simulink model "bimanual_Diedrichsen"  (Simulink 8.1)
settings: Solver=ode4  SolverMode=SingleTasking  StartTime=0.0  StopTime=inf  FixedStep=0.0005  RelTol=1e-3
model workspace (MAT data in the model file):
  col_x = 1
  col_y = 2
  COL_VRAD = 3
  COL_LRAD = 4
  COL_FRAD = 5
  COL_COLOUR = 6
  COL_GOOD_COLOUR = 7
  COL_SLOW_COLOUR = 8
  COL_MISSED_COLOUR = 9
  COL_VY_ON_FX1 = 1
  COL_VY_ON_FX2 = 2
  COL_START_TARGET = 1
  COL_END_TARGET = 2
  COL_LOAD = 3
  COL_CURSOR_SELECTION = 4
  COL_1ST_TARGET_WAIT = 5
  COL_RANDOM_WAIT = 6
  COL_MAX_REACH_TIME = 7
  COL_2ND_TARGET_WAIT = 8
  COL_POST_TRIAL_DELAY = 9
  COL_HAND_FEEDBACK = 10
  E_STAY_CENTER = 2
  E_TARGET_ON = 3
  E_HOLD_AT_TARGET = 5
  E_HAND_FDBK_OFF = 11
  BKIN_STEP_TIME : num (value not decoded)
StartFcn:
  |  warndlg('Dexterit-E models cannot run under simulation. Please compile your model and run it from within Dexterit-E.');set_param(bdroot,'SimulationCommand','stop')
undefined symbols (not defined in the file or in its folder): slselsubs
libraries: Video x3, General x3, KINARM_EP_loads x3, KINARM_general x2, KINARM_loads x2, xpclib x1
(part 1 of 3)
CloseFcn:
  | rtwprivate ssgencode ModelCloseRequest b2lab2d
settings Model: Creator=Chris Grebeldinger  LastModifiedBy=dmclean  ModifiedComment=chris -- Wed Feb 16 09:18:30 2005 -- Version 1.1384  ModifiedHistory=Feb 16/05 - Add error repeat, add offset ramp  ExtModeArmWhenConnect=off  ExtModeLogAll=off  BufferReuse=off
settings DataIOCC: LimitDataPoints=off  SaveOutput=off  SaveTime=off  SignalLoggingName=sigsOut
settings OptimizationCC: BlockReduction=off  BooleanDataType=off  OptimizeBlockIOStorage=off  BufferReuse=off  ExpressionFolding=off  FoldNonRolledExpr=off  LocalBlockOutputs=off  InitFltsAndDblsToZero=on
settings DebuggingCC: SaveWithParameterizedLinksMsg=none  SignalResolutionControl=TryResolveAllWithWarning  SolverPrmCheckMsg=none  MultiTaskDSMMsg=warning  MultiTaskCondExecSysMsg=none  StrictBusMsg=None
settings HardwareCC: ProdIntDivRoundTo=Zero  ProdEndianess=LittleEndian  ProdHWDeviceType=Generic->32-bit x86 compatible  TargetHWDeviceType=32-bit Generic
settings SFSimCC: SimParseCustomCode=off
settings RTWCC: SystemTargetFile=xpctarget.tlc  TemplateMakefile=xpc_default_tmf  Description=xPC Target  ProcessScript=xpctarget_make_rtw_hook  IncludeERTFirstTime=on  RTWCompilerOptimization=On
settings CodeAppCC: MaxIdLength=63
settings xpcTargetCC: TargetFcnLib=ansi_tfl_tmw.mat  CodeReplacementLibrary=XPC_BLAS  ParMdlRefBuildCompliant=on  ConcurrentExecutionCompliant=on  CombineSignalStateStructs=off  MATLABClassNameForMDSCustomization=xpcAperiodicCustomization  GRTInterface=on  GenerateAllocFcn=off  xPCTaskExecutionProfile=off  xPCRL32EventNumber=5000  xPCisDownloadable=off  xPCLoadParamSetFile=off  xPCConcurrentTasks=off  xPCEnableSFAnimation=off

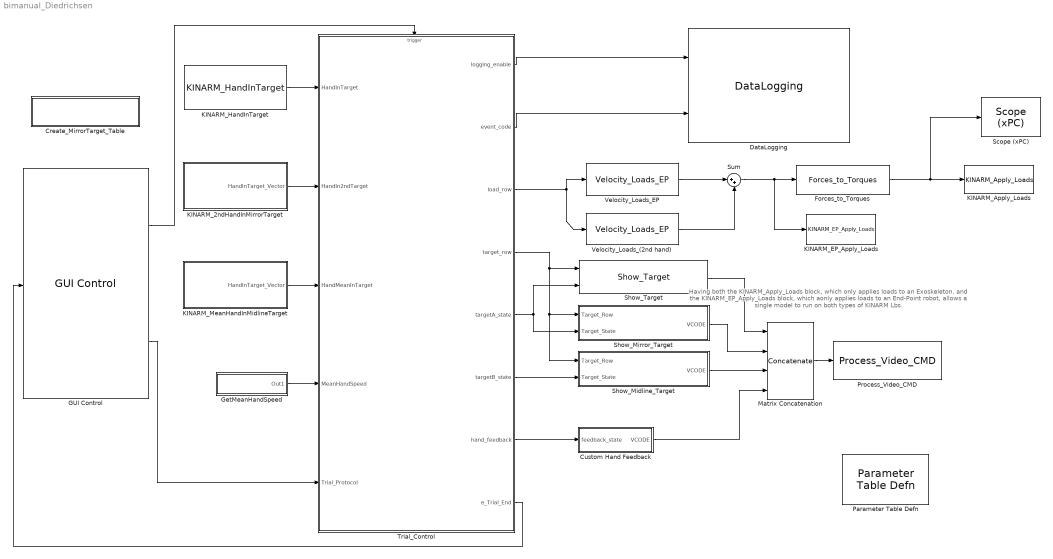
== system bimanual_Diedrichsen ==
  note: Having both the KINARM_Apply_Loads block, which only
      | applies loads to an Exoskeleton, and the KINARM_EP_Apply_Loads
      |  block, which aonly applies loads to an End-Point robot, allows
      | a single model to run on both types of KINARM Lbs.
  Create_MirrorTarget_Table : Subsystem
  Custom Hand Feedback : Subsystem
  DataLogging : General/DataLogging  log_event_codes=on  log_analog_inputs=off
      link override Poll KINARM/EPTorqueCMD: GotoTag=KINARMEPTorqueCMD
      link override Poll KINARM/TorqueCMD: GotoTag=KINARMTorqueCMD
  Forces_to_Torques : KINARM_loads/Forces_to_Torques
  GUI Control : General/GUI Control  target_type_str=Circle  Target_Type=1  XYcols=[1 2]  Vcols=3  Lcols=4  indices_padding=[0 0 0 0;0 0 0 0]  task_version=1.0  show_repeat_trial_flag=off
  GetMeanHandSpeed : Subsystem
  KINARM_2ndHandInMirrorTarget : Subsystem  AncestorBlock=KINARM_general/KINARM_HandInTarget  mask(KINARM_HandInTarget){use_dominant_hand=off, target_type=Circle, num_states=1, attribcol1=4, attribcol2=4, attribcol3=5, attribcol4=6}
      mask prompts: use_dominant_hand "Dominant Hand?"; target_type "Type of Target"; num_states "Number of Target States"; attribcol1 "State 1 Target Table Column(s)"; attribcol2 "State 2 Target Table Column(s)"; attribcol3 "State 3 Target Table Column(s)"; attribcol4 "State 4 Target Table Column(s)"
      mask help: This block returns a vector or array corresponding to the Target_Table rows indicating whether the specified hand is in (=1) or out (=0) of each of the targets.
      mask init:
      | num_states=str2num(get_param(gcb, 'num_states'));
      | columntext='(columns: ';
      | 
      | for i=1:num_states
      | 	varname=['attribcol' num2str(i)];
      | 	if i>1
      | 		columntext=[columntext, '; '];
      | 	end
      | 	columntext=[columntext, get_param(gcb, varname)];
      | end
      | columntext=strvcat([columntext ')'],' ', ' ');
      | 
      | output_block=char(find_system(gcb,'LookUnderMasks','all','FollowLinks','on','SearchDepth',1,'BlockType','Outport'));
      | outputname=get_param(output_block,'Name');
      | 
      | % Select only the desired states for output. The output port is also renamed to reflect 
      | % whether the output is a vector (in the case of a single state) or an array (of vectors, 
      | % one for each of multiple states).
      | if num_states == 1
      | 	set_param([gcb '/Selected States'], 'Value', '[1]');
      | 	set_param(output_block, 'Name', 'HandInTarget_Vector');
      | elseif num_states == 2
      | 	set_param([gcb '/Selected States'], 'Value', '[1,2]');
      | 	set_param(output_block, 'Name', 'HandInTarget_Array');
      | elseif num_states == 3
      | 	set_param([gcb '/Selected States'], 'Value', '[1,2,3]');
      | 	set_param(output_block, 'Name', 'HandInTarget_Array');
      | else
      | 	set_param([gcb '/Selected States'], 'Value', '[1,2,3,4]');
      | 	set_param(output_block, 'Name', 'HandInTarget_Array');
      | end
      mask Help:
      | Used to determine if the hand (finger-tip) is in any of the targets in the Target_Table.
      | <P>
      | <B><I>Use of this block requires that the DataLogging block (General library) be set to log KINARM data.</I></B>
      | 
      | <H2>Library </H2>
      | KINARM_general (sub-library)
      | 
      | <H2>Description </H2>
      | This block returns a vector or array corresponding to the Target_Table rows indicating whether the specified hand (i.e. finger-tip) is in or out of each of the targets.  Each element in the output vector or output array will be either a 0 (hand not in target) or a 1 (hand in target).
      | <P>
      | A vector is returned if only one target state is specified in each target row (see Parameters and Dialog Box), with each index of the vector corresponding to a row in the target table.  An array is returned if more than one target state is specified in a target row, with each row of the array corresponding to a target row and each column corresponding to the nth target state specified in each target row.
      | <P>
      | The output vector or array is typically used by a stateflow chart to affect behavior of the system.  Because this block returns hand-in-target information for all targets in the target table, multiple targets can be monitored at once (i.e. the stateflow chart could have certain transitions that occur if the hand is in one target and other transitions if it is in a different target).  Likewise, because this block returns hand-in-target information for multiple states of a single target, those multiple states can be monitored simultaneously.
      | <P>
      | Because the KINARM_HandInTarget block returns information for only one hand, two copies of this block are required if information for both hands is desired.
      | <P>
      | 
      | <H2>Parameters and Dialog Box</H2>
      | <B>Dominant Hand?:</B> this box determines which hand is used by this block : dominant hand position (checked box) or the non-dominant hand position (unchecked box).  (Note: if the end-user wants to know about both the dominant hand and the non-dominant hand, then 2 separate copies of this block are requried, one for each hand.)
      | <P>
      | <B>Type of Target:</B> Enter the type of target specified in the target table:
      | <P>
      | <B>Number of Target States:</B> Enter the number of target states specified in each target row.  Up to four target states are allowed per target row.
      | <P>
      | <B>State <n> Target Table Columns:</B> Enter the columns in the Target Table that specify the relevant target attributes.  Do this for each target state.
      | For a circle, enter the columns corresponding to logical radius (e.g. 4)
      | <BR>For an ellipse, enter the columns corresponding to major radius, minor radius, rotation angle (e.g. [4, 5, 6]).
      | <BR>For a rectangle, enter the columns corresponding to length, height, and rotation angle (e.g. [4, 5, 6]).
      | <BR>For a line, enter the columns corresponding to stroke width, endpoint in x, and endpoint in y (e.g. [3, 4, 5]).
      | <BR>For a triangle, enter the columns corresponding to length, height, peak offset, and rotation angle (e.g. [4, 5, 6, 7]).
      | 
      | <H2>Examples</H2>
      | <B>Example 1.</B>  Suppose a target row will be used to define 1 state for a circle type target and the radius of the visual target is the same radius to be used for determination of hand-in-target.  The related Target Table column is: column 6 = radius.  For this example, "State 1 Target Table Columns" would equal [6].
      | <P>
      | 
      | <B>Example 2.</B>  Suppose a target row will be used to define 1 state for a circle type target, but the radius of the visual target will be different than the radius to be used for determination of hand-in-target.  This option allows independent control over the size of the visual target versus the accuracy needed to be considered "in the target".  The related Target Table columns are: column 6 = radius1 (i.e. radius to target to be drawn); column 7 = radius2 (i.e. radius to be used for hand-in-target) .  For this example, "State 1 Target Table Columns" would equal [7].
      | <P>
      | <B>Example 3.</B>  Suppose a target row will be used to define 2 states for a circle type target, where the radius of the visual target will be a constant, but depending on the state of the system, one of 2 other and different radii will be used for determination of hand-in-target.  The related Target Table columns are: column 6 = radius1 (i.e. radius to target to be drawn); column 7 = radius2 (i.e. radius to be used for hand-in-target for state 1); column 8 = radius3 (i.e. radius to be used for hand-in-target for state 2).  For this example, "State 1 Target Table Columns" would equal [7], while "State 2 Target Table Columns" would equal [8].
      | <P>
      | 
      | <H2>Related Blocks </H2>
      | DataLogging
      mask TypeOptions target_type: Circle | Ellipse | Rectangle | Line | Triangle
      mask Callback target_type:
      | target_type=get_param(gcb, 'target_type');
      | attribcol1=[str2num(get_param(gcb, 'attribcol1')) 0 0 0 0 0 0];
      | attribcol2=[str2num(get_param(gcb, 'attribcol2')) 0 0 0 0 0 0];
      | attribcol3=[str2num(get_param(gcb, 'attribcol3')) 0 0 0 0 0 0];
      | attribcol4=[str2num(get_param(gcb, 'attribcol4')) 0 0 0 0 0 0];
      | switch target_type(1:3)
      | 	case 'Cir'
      | 		numcol=1;
      | 	case 'Ell'
      | 		numcol=3;
      |     case 'Rec'
      |         numcol=3;
      |     case 'Lin'
      |         numcol=3;
      |     case 'Tri'
      |         numcol=4;
      | 	otherwise
      | 		numcol=1;
      | end
      | if numcol==1
      | 	set_param(gcb, 'attribcol1', num2str(attribcol1(1)));
      | 	set_param(gcb, 'attribcol2', num2str(attribcol2(1)));
      | 	set_param(gcb, 'attribcol3', num2str(attribcol3(1)));
      | 	set_param(gcb, 'attribcol4', num2str(attribcol4(1)));
      | else
      | 	set_param(gcb, 'attribcol1', ['[' num2str(attribcol1(1:numcol)) ']']);
      | 	set_param(gcb, 'attribcol2', ['[' num2str(attribcol2(1:numcol)) ']']);
      | 	set_param(gcb, 'attribcol3', ['[' num2str(attribcol3(1:numcol)) ']']);
      | 	set_param(gcb, 'attribcol4', ['[' num2str(attribcol4(1:numcol)) ']']);
      | end
      mask TypeOptions num_states: 1 | 2 | 3 | 4
      mask Callback num_states:
      | num_states = str2num(get_param(gcb, 'num_states'));
      | vis = get_param(gcb, 'MaskVisibilities');
      | 
      | % Select only the desired states for output. The output port is also renamed to reflect
      | % whether the output is a vector (in the case of a single state) or an array (of vectors,
      | % one for each of multiple states).
      | output_block=char(find_system(gcb, 'LookUnderMasks', 'all', 'FollowLinks', 'on', 'SearchDepth', 1, 'BlockType', 'Outport'));
      | 
      | if num_states == 1
      | 	set_param([gcb '/Selected States'], 'Value', '[1]');
      | 	set_param(output_block, 'Name', 'HandInTarget_Vector');
      | 	vis{5} = 'off';
      | 	vis{6} = 'off';
      | 	vis{7} = 'off';
      | elseif num_states == 2
      | 	set_param([gcb '/Selected States'], 'Value', '[1,2]');
      | 	set_param(output_block, 'Name', 'HandInTarget_Array');
      | 	vis{5} = 'on';
      | 	vis{6} = 'off';
      | 	vis{7} = 'off';
      | elseif num_states == 3
      | 	set_param([gcb '/Selected States'], 'Value', '[1,2,3]');
      | 	set_param(output_block, 'Name','HandInTarget_Array');
      | 	vis{5} = 'on';
      | 	vis{6} = 'on';
      | 	vis{7} = 'off';
      | else
      | 	set_param([gcb '/Selected States'], 'Value', '[1,2,3,4]');
      | 	set_param(output_block, 'Name', 'HandInTarget_Array');
      | 	vis{5} = 'on';
      | 	vis{6} = 'on';
      | 	vis{7} = 'on';
      | end
      | set_param(gcb, 'MaskVisibilities', vis);
      | 
      | target_type=get_param(gcb, 'target_type');
      | attribcol1=[str2num(get_param(gcb, 'attribcol1')) 0 0 0 0 0 0];
      | attribcol2=[str2num(get_param(gcb, 'attribcol2')) 0 0 0 0 0 0];
      | attribcol3=[str2num(get_param(gcb, 'attribcol3')) 0 0 0 0 0 0];
      | attribcol4=[str2num(get_param(gcb, 'attribcol4')) 0 0 0 0 0 0];
      | switch target_type(1:3)
      | 	case 'Cir'
      | 		numcol=1;
      | 	case 'Ell'
      | 		numcol=3;
      |     case 'Rec'
      |         numcol=3;
      |     case 'Lin'
      |         numcol=3;
      |     case 'Tri'
      |         numcol=4;
      | 	otherwise
      | 		numcol=1;
      | end
      | if numcol==1
      | 	set_param(gcb, 'attribcol1', num2str(attribcol1(1)));
      | 	set_param(gcb, 'attribcol2', num2str(attribcol2(1)));
      | 	set_param(gcb, 'attribcol3', num2str(attribcol3(1)));
      | 	set_param(gcb, 'attribcol4', num2str(attribcol4(1)));
      | else
      | 	set_param(gcb, 'attribcol1', ['[' num2str(attribcol1(1:numcol)) ']']);
      | 	set_param(gcb, 'attribcol2', ['[' num2str(attribcol2(1:numcol)) ']']);
      | 	set_param(gcb, 'attribcol3', ['[' num2str(attribcol3(1:numcol)) ']']);
      | 	set_param(gcb, 'attribcol4', ['[' num2str(attribcol4(1:numcol)) ']']);
      | end
      mask Callback attribcol1:
      | target_type=get_param(gcb, 'target_type');
      | attribcol1=[str2num(get_param(gcb, 'attribcol1')) 0 0 0 0 0 0];
      | attribcol2=[str2num(get_param(gcb, 'attribcol2')) 0 0 0 0 0 0];
      | attribcol3=[str2num(get_param(gcb, 'attribcol3')) 0 0 0 0 0 0];
      | attribcol4=[str2num(get_param(gcb, 'attribcol4')) 0 0 0 0 0 0];
      | switch target_type(1:3)
      | 	case 'Cir'
      | 		numcol=1;
      | 	case 'Ell'
      | 		numcol=3;
      |     case 'Rec'
      |         numcol=3;
      |     case 'Lin'
      |         numcol=3;
      |     case 'Tri'
      |         numcol=4;
      | 	otherwise
      | 		numcol=1;
      | end
      | if numcol==1
      | 	set_param(gcb, 'attribcol1', num2str(attribcol1(1)));
      | 	set_param(gcb, 'attribcol2', num2str(attribcol2(1)));
      | 	set_param(gcb, 'attribcol3', num2str(attribcol3(1)));
      | 	set_param(gcb, 'attribcol4', num2str(attribcol4(1)));
      | else
      | 	set_param(gcb, 'attribcol1', ['[' num2str(attribcol1(1:numcol)) ']']);
      | 	set_param(gcb, 'attribcol2', ['[' num2str(attribcol2(1:numcol)) ']']);
      | 	set_param(gcb, 'attribcol3', ['[' num2str(attribcol3(1:numcol)) ']']);
      | 	set_param(gcb, 'attribcol4', ['[' num2str(attribcol4(1:numcol)) ']']);
      | end
      mask Callback attribcol2:
      | target_type=get_param(gcb, 'target_type');
      | attribcol1=[str2num(get_param(gcb, 'attribcol1')) 0 0 0 0 0 0];
      | attribcol2=[str2num(get_param(gcb, 'attribcol2')) 0 0 0 0 0 0];
      | attribcol3=[str2num(get_param(gcb, 'attribcol3')) 0 0 0 0 0 0];
      | attribcol4=[str2num(get_param(gcb, 'attribcol4')) 0 0 0 0 0 0];
      | switch target_type(1:3)
      | 	case 'Cir'
      | 		numcol=1;
      | 	case 'Ell'
      | 		numcol=3;
      |     case 'Rec'
      |         numcol=3;
      |     case 'Lin'
      |         numcol=3;
      |     case 'Tri'
      |         numcol=4;
      | 	otherwise
      | 		numcol=1;
      | end
      | if numcol==1
      | 	set_param(gcb, 'attribcol1', num2str(attribcol1(1)));
      | 	set_param(gcb, 'attribcol2', num2str(attribcol2(1)));
      | 	set_param(gcb, 'attribcol3', num2str(attribcol3(1)));
      | 	set_param(gcb, 'attribcol4', num2str(attribcol4(1)));
      | else
      | 	set_param(gcb, 'attribcol1', ['[' num2str(attribcol1(1:numcol)) ']']);
      | 	set_param(gcb, 'attribcol2', ['[' num2str(attribcol2(1:numcol)) ']']);
      | 	set_param(gcb, 'attribcol3', ['[' num2str(attribcol3(1:numcol)) ']']);
      | 	set_param(gcb, 'attribcol4', ['[' num2str(attribcol4(1:numcol)) ']']);
      | end
      mask Callback attribcol3:
      | target_type=get_param(gcb, 'target_type');
      | attribcol1=[str2num(get_param(gcb, 'attribcol1')) 0 0 0 0 0 0];
      | attribcol2=[str2num(get_param(gcb, 'attribcol2')) 0 0 0 0 0 0];
      | attribcol3=[str2num(get_param(gcb, 'attribcol3')) 0 0 0 0 0 0];
      | attribcol4=[str2num(get_param(gcb, 'attribcol4')) 0 0 0 0 0 0];
      | switch target_type(1:3)
      | 	case 'Cir'
      | 		numcol=1;
      | 	case 'Ell'
      | 		numcol=3;
      |     case 'Rec'
      |         numcol=3;
      |     case 'Lin'
      |         numcol=3;
      |     case 'Tri'
      |         numcol=4;
      | 	otherwise
      | 		numcol=1;
      | end
      | if numcol==1
      | 	set_param(gcb, 'attribcol1', num2str(attribcol1(1)));
      | 	set_param(gcb, 'attribcol2', num2str(attribcol2(1)));
      | 	set_param(gcb, 'attribcol3', num2str(attribcol3(1)));
      | 	set_param(gcb, 'attribcol4', num2str(attribcol4(1)));
      | else
      | 	set_param(gcb, 'attribcol1', ['[' num2str(attribcol1(1:numcol)) ']']);
      | 	set_param(gcb, 'attribcol2', ['[' num2str(attribcol2(1:numcol)) ']']);
      | 	set_param(gcb, 'attribcol3', ['[' num2str(attribcol3(1:numcol)) ']']);
      | 	set_param(gcb, 'attribcol4', ['[' num2str(attribcol4(1:numcol)) ']']);
      | end
      mask Callback attribcol4:
      | target_type=get_param(gcb, 'target_type');
      | attribcol1=[str2num(get_param(gcb, 'attribcol1')) 0 0 0 0 0 0];
      | attribcol2=[str2num(get_param(gcb, 'attribcol2')) 0 0 0 0 0 0];
      | attribcol3=[str2num(get_param(gcb, 'attribcol3')) 0 0 0 0 0 0];
      | attribcol4=[str2num(get_param(gcb, 'attribcol4')) 0 0 0 0 0 0];
      | switch target_type(1:3)
      | 	case 'Cir'
      | 		numcol=1;
      | 	case 'Ell'
      | 		numcol=3;
      |     case 'Rec'
      |         numcol=3;
      |     case 'Lin'
      |         numcol=3;
      |     case 'Tri'
      |         numcol=4;
      | 	otherwise
      | 		numcol=1;
      | end
      | if numcol==1
      | 	set_param(gcb, 'attribcol1', num2str(attribcol1(1)));
      | 	set_param(gcb, 'attribcol2', num2str(attribcol2(1)));
      | 	set_param(gcb, 'attribcol3', num2str(attribcol3(1)));
      | 	set_param(gcb, 'attribcol4', num2str(attribcol4(1)));
      | else
      | 	set_param(gcb, 'attribcol1', ['[' num2str(attribcol1(1:numcol)) ']']);
      | 	set_param(gcb, 'attribcol2', ['[' num2str(attribcol2(1:numcol)) ']']);
      | 	set_param(gcb, 'attribcol3', ['[' num2str(attribcol3(1:numcol)) ']']);
      | 	set_param(gcb, 'attribcol4', ['[' num2str(attribcol4(1:numcol)) ']']);
      | end
      mask Display:
      | disp(columntext)
      | port_label('output',1,outputname)
  KINARM_Apply_Loads : KINARM_loads/KINARM_Apply_Loads  up_duration=50  down_duration=50  max_torque=13
  KINARM_EP_Apply_Loads : KINARM_EP_loads/KINARM_EP_Apply_Loads  up_duration=1500  down_duration=1500  max_force=60
  KINARM_HandInTarget : KINARM_general/KINARM_HandInTarget  use_dominant_hand=on  target_type=Circle  num_states=1  attribcol1=[4]  attribcol2=[4]  attribcol3=[5]  attribcol4=[6]  attribcol5=[0]
  KINARM_MeanHandInMidlineTarget : Subsystem  AncestorBlock=KINARM_general/KINARM_HandInTarget  mask(KINARM_HandInTarget){use_dominant_hand=off, target_type=Circle, num_states=1, attribcol1=4, attribcol2=4, attribcol3=5, attribcol4=6}
      mask prompts: use_dominant_hand "Dominant Hand?"; target_type "Type of Target"; num_states "Number of Target States"; attribcol1 "State 1 Target Table Column(s)"; attribcol2 "State 2 Target Table Column(s)"; attribcol3 "State 3 Target Table Column(s)"; attribcol4 "State 4 Target Table Column(s)"
      mask help: This block returns a vector or array corresponding to the Target_Table rows indicating whether the specified hand is in (=1) or out (=0) of each of the targets.
      mask init: same as bimanual_Diedrichsen/KINARM_2ndHandInMirrorTarget
      mask Help:
      | Used to determine if the hand (finger-tip) is in any of the targets in the Target_Table.
      | <P>
      | <B><I>Use of this block requires that the DataLogging block (General library) be set to log KINARM data.</I></B>
      | 
      | <H2>Library </H2>
      | KINARM_general (sub-library)
      | 
      | <H2>Description </H2>
      | This block returns a vector or array corresponding to the Target_Table rows indicating whether the specified hand (i.e. finger-tip) is in or out of each of the targets.  Each element in the output vector or output array will be either a 0 (hand not in target) or a 1 (hand in target).
      | <P>
      | A vector is returned if only one target state is specified in each target row (see Parameters and Dialog Box), with each index of the vector corresponding to a row in the target table.  An array is returned if more than one target state is specified in a target row, with each row of the array corresponding to a target row and each column corresponding to the nth target state specified in each target row.
      | <P>
      | The output vector or array is typically used by a stateflow chart to affect behavior of the system.  Because this block returns hand-in-target information for all targets in the target table, multiple targets can be monitored at once (i.e. the stateflow chart could have certain transitions that occur if the hand is in one target and other transitions if it is in a different target).  Likewise, because this block returns hand-in-target information for multiple states of a single target, those multiple states can be monitored simultaneously.
      | <P>
      | Because the KINARM_HandInTarget block returns information for only one hand, two copies of this block are required if information for both hands is desired.
      | <P>
      | 
      | <H2>Parameters and Dialog Box</H2>
      | <B>Dominant Hand?:</B> this box determines which hand is used by this block : dominant hand position (checked box) or the non-dominant hand position (unchecked box).  (Note: if the end-user wants to know about both the dominant hand and the non-dominant hand, then 2 separate copies of this block are requried, one for each hand.)
      | <P>
      | <B>Type of Target:</B> Enter the type of target specified in the target table:
      | <P>
      | <B>Number of Target States:</B> Enter the number of target states specified in each target row.  Up to four target states are allowed per target row.
      | <P>
      | <B>State <n> Target Table Columns:</B> Enter the columns in the Target Table that specify the relevant target attributes.  Do this for each target state.
      | For a circle, enter the columns corresponding to logical radius (e.g. 4)
      | <BR>For an ellipse, enter the columns corresponding to major radius, minor radius, rotation angle (e.g. [4, 5, 6]).
      | <BR>For a rectangle, enter the columns corresponding to length, height, and rotation angle (e.g. [4, 5, 6]).
      | <BR>For a line, enter the columns corresponding to stroke width, endpoint in x, and endpoint in y (e.g. [3, 4, 5]).
      | <BR>For a triangle, enter the columns corresponding to length, height, peak offset, and rotation angle (e.g. [4, 5, 6, 7]).
      | 
      | <H2>Examples</H2>
      | <B>Example 1.</B>  Suppose a target row will be used to define 1 state for a circle type target and the radius of the visual target is the same radius to be used for determination of hand-in-target.  The related Target Table column is: column 6 = radius.  For this example, "State 1 Target Table Columns" would equal [6].
      | <P>
      | 
      | <B>Example 2.</B>  Suppose a target row will be used to define 1 state for a circle type target, but the radius of the visual target will be different than the radius to be used for determination of hand-in-target.  This option allows independent control over the size of the visual target versus the accuracy needed to be considered "in the target".  The related Target Table columns are: column 6 = radius1 (i.e. radius to target to be drawn); column 7 = radius2 (i.e. radius to be used for hand-in-target) .  For this example, "State 1 Target Table Columns" would equal [7].
      | <P>
      | <B>Example 3.</B>  Suppose a target row will be used to define 2 states for a circle type target, where the radius of the visual target will be a constant, but depending on the state of the system, one of 2 other and different radii will be used for determination of hand-in-target.  The related Target Table columns are: column 6 = radius1 (i.e. radius to target to be drawn); column 7 = radius2 (i.e. radius to be used for hand-in-target for state 1); column 8 = radius3 (i.e. radius to be used for hand-in-target for state 2).  For this example, "State 1 Target Table Columns" would equal [7], while "State 2 Target Table Columns" would equal [8].
      | <P>
      | 
      | <H2>Related Blocks </H2>
      | DataLogging
      mask TypeOptions target_type: Circle | Ellipse | Rectangle | Line | Triangle
      mask Callback target_type:
      | target_type=get_param(gcb, 'target_type');
      | attribcol1=[str2num(get_param(gcb, 'attribcol1')) 0 0 0 0 0 0];
      | attribcol2=[str2num(get_param(gcb, 'attribcol2')) 0 0 0 0 0 0];
      | attribcol3=[str2num(get_param(gcb, 'attribcol3')) 0 0 0 0 0 0];
      | attribcol4=[str2num(get_param(gcb, 'attribcol4')) 0 0 0 0 0 0];
      | switch target_type(1:3)
      | 	case 'Cir'
      | 		numcol=1;
      | 	case 'Ell'
      | 		numcol=3;
      |     case 'Rec'
      |         numcol=3;
      |     case 'Lin'
      |         numcol=3;
      |     case 'Tri'
      |         numcol=4;
      | 	otherwise
      | 		numcol=1;
      | end
      | if numcol==1
      | 	set_param(gcb, 'attribcol1', num2str(attribcol1(1)));
      | 	set_param(gcb, 'attribcol2', num2str(attribcol2(1)));
      | 	set_param(gcb, 'attribcol3', num2str(attribcol3(1)));
      | 	set_param(gcb, 'attribcol4', num2str(attribcol4(1)));
      | else
      | 	set_param(gcb, 'attribcol1', ['[' num2str(attribcol1(1:numcol)) ']']);
      | 	set_param(gcb, 'attribcol2', ['[' num2str(attribcol2(1:numcol)) ']']);
      | 	set_param(gcb, 'attribcol3', ['[' num2str(attribcol3(1:numcol)) ']']);
      | 	set_param(gcb, 'attribcol4', ['[' num2str(attribcol4(1:numcol)) ']']);
      | end
      mask TypeOptions num_states: 1 | 2 | 3 | 4
      mask Callback num_states:
      | num_states = str2num(get_param(gcb, 'num_states'));
      | vis = get_param(gcb, 'MaskVisibilities');
      | 
      | % Select only the desired states for output. The output port is also renamed to reflect
      | % whether the output is a vector (in the case of a single state) or an array (of vectors,
      | % one for each of multiple states).
      | output_block=char(find_system(gcb, 'LookUnderMasks', 'all', 'FollowLinks', 'on', 'SearchDepth', 1, 'BlockType', 'Outport'));
      | 
      | if num_states == 1
      | 	set_param([gcb '/Selected States'], 'Value', '[1]');
      | 	set_param(output_block, 'Name', 'HandInTarget_Vector');
      | 	vis{5} = 'off';
      | 	vis{6} = 'off';
      | 	vis{7} = 'off';
      | elseif num_states == 2
      | 	set_param([gcb '/Selected States'], 'Value', '[1,2]');
      | 	set_param(output_block, 'Name', 'HandInTarget_Array');
      | 	vis{5} = 'on';
      | 	vis{6} = 'off';
      | 	vis{7} = 'off';
      | elseif num_states == 3
      | 	set_param([gcb '/Selected States'], 'Value', '[1,2,3]');
      | 	set_param(output_block, 'Name','HandInTarget_Array');
      | 	vis{5} = 'on';
      | 	vis{6} = 'on';
      | 	vis{7} = 'off';
      | else
      | 	set_param([gcb '/Selected States'], 'Value', '[1,2,3,4]');
      | 	set_param(output_block, 'Name', 'HandInTarget_Array');
      | 	vis{5} = 'on';
      | 	vis{6} = 'on';
      | 	vis{7} = 'on';
      | end
      | set_param(gcb, 'MaskVisibilities', vis);
      | 
      | target_type=get_param(gcb, 'target_type');
      | attribcol1=[str2num(get_param(gcb, 'attribcol1')) 0 0 0 0 0 0];
      | attribcol2=[str2num(get_param(gcb, 'attribcol2')) 0 0 0 0 0 0];
      | attribcol3=[str2num(get_param(gcb, 'attribcol3')) 0 0 0 0 0 0];
      | attribcol4=[str2num(get_param(gcb, 'attribcol4')) 0 0 0 0 0 0];
      | switch target_type(1:3)
      | 	case 'Cir'
      | 		numcol=1;
      | 	case 'Ell'
      | 		numcol=3;
      |     case 'Rec'
      |         numcol=3;
      |     case 'Lin'
      |         numcol=3;
      |     case 'Tri'
      |         numcol=4;
      | 	otherwise
      | 		numcol=1;
      | end
      | if numcol==1
      | 	set_param(gcb, 'attribcol1', num2str(attribcol1(1)));
      | 	set_param(gcb, 'attribcol2', num2str(attribcol2(1)));
      | 	set_param(gcb, 'attribcol3', num2str(attribcol3(1)));
      | 	set_param(gcb, 'attribcol4', num2str(attribcol4(1)));
      | else
      | 	set_param(gcb, 'attribcol1', ['[' num2str(attribcol1(1:numcol)) ']']);
      | 	set_param(gcb, 'attribcol2', ['[' num2str(attribcol2(1:numcol)) ']']);
      | 	set_param(gcb, 'attribcol3', ['[' num2str(attribcol3(1:numcol)) ']']);
      | 	set_param(gcb, 'attribcol4', ['[' num2str(attribcol4(1:numcol)) ']']);
      | end
      mask Callback attribcol1:
      | target_type=get_param(gcb, 'target_type');
      | attribcol1=[str2num(get_param(gcb, 'attribcol1')) 0 0 0 0 0 0];
      | attribcol2=[str2num(get_param(gcb, 'attribcol2')) 0 0 0 0 0 0];
      | attribcol3=[str2num(get_param(gcb, 'attribcol3')) 0 0 0 0 0 0];
      | attribcol4=[str2num(get_param(gcb, 'attribcol4')) 0 0 0 0 0 0];
      | switch target_type(1:3)
      | 	case 'Cir'
      | 		numcol=1;
      | 	case 'Ell'
      | 		numcol=3;
      |     case 'Rec'
      |         numcol=3;
      |     case 'Lin'
      |         numcol=3;
      |     case 'Tri'
      |         numcol=4;
      | 	otherwise
      | 		numcol=1;
      | end
      | if numcol==1
      | 	set_param(gcb, 'attribcol1', num2str(attribcol1(1)));
      | 	set_param(gcb, 'attribcol2', num2str(attribcol2(1)));
      | 	set_param(gcb, 'attribcol3', num2str(attribcol3(1)));
      | 	set_param(gcb, 'attribcol4', num2str(attribcol4(1)));
      | else
      | 	set_param(gcb, 'attribcol1', ['[' num2str(attribcol1(1:numcol)) ']']);
      | 	set_param(gcb, 'attribcol2', ['[' num2str(attribcol2(1:numcol)) ']']);
      | 	set_param(gcb, 'attribcol3', ['[' num2str(attribcol3(1:numcol)) ']']);
      | 	set_param(gcb, 'attribcol4', ['[' num2str(attribcol4(1:numcol)) ']']);
      | end
      mask Callback attribcol2:
      | target_type=get_param(gcb, 'target_type');
      | attribcol1=[str2num(get_param(gcb, 'attribcol1')) 0 0 0 0 0 0];
      | attribcol2=[str2num(get_param(gcb, 'attribcol2')) 0 0 0 0 0 0];
      | attribcol3=[str2num(get_param(gcb, 'attribcol3')) 0 0 0 0 0 0];
      | attribcol4=[str2num(get_param(gcb, 'attribcol4')) 0 0 0 0 0 0];
      | switch target_type(1:3)
      | 	case 'Cir'
      | 		numcol=1;
      | 	case 'Ell'
      | 		numcol=3;
      |     case 'Rec'
      |         numcol=3;
      |     case 'Lin'
      |         numcol=3;
      |     case 'Tri'
      |         numcol=4;
      | 	otherwise
      | 		numcol=1;
      | end
      | if numcol==1
      | 	set_param(gcb, 'attribcol1', num2str(attribcol1(1)));
      | 	set_param(gcb, 'attribcol2', num2str(attribcol2(1)));
      | 	set_param(gcb, 'attribcol3', num2str(attribcol3(1)));
      | 	set_param(gcb, 'attribcol4', num2str(attribcol4(1)));
      | else
      | 	set_param(gcb, 'attribcol1', ['[' num2str(attribcol1(1:numcol)) ']']);
      | 	set_param(gcb, 'attribcol2', ['[' num2str(attribcol2(1:numcol)) ']']);
      | 	set_param(gcb, 'attribcol3', ['[' num2str(attribcol3(1:numcol)) ']']);
      | 	set_param(gcb, 'attribcol4', ['[' num2str(attribcol4(1:numcol)) ']']);
      | end
      mask Callback attribcol3:
      | target_type=get_param(gcb, 'target_type');
      | attribcol1=[str2num(get_param(gcb, 'attribcol1')) 0 0 0 0 0 0];
      | attribcol2=[str2num(get_param(gcb, 'attribcol2')) 0 0 0 0 0 0];
      | attribcol3=[str2num(get_param(gcb, 'attribcol3')) 0 0 0 0 0 0];
      | attribcol4=[str2num(get_param(gcb, 'attribcol4')) 0 0 0 0 0 0];
      | switch target_type(1:3)
      | 	case 'Cir'
      | 		numcol=1;
      | 	case 'Ell'
      | 		numcol=3;
      |     case 'Rec'
      |         numcol=3;
      |     case 'Lin'
      |         numcol=3;
      |     case 'Tri'
      |         numcol=4;
      | 	otherwise
      | 		numcol=1;
      | end
      | if numcol==1
      | 	set_param(gcb, 'attribcol1', num2str(attribcol1(1)));
      | 	set_param(gcb, 'attribcol2', num2str(attribcol2(1)));
      | 	set_param(gcb, 'attribcol3', num2str(attribcol3(1)));
      | 	set_param(gcb, 'attribcol4', num2str(attribcol4(1)));
      | else
      | 	set_param(gcb, 'attribcol1', ['[' num2str(attribcol1(1:numcol)) ']']);
      | 	set_param(gcb, 'attribcol2', ['[' num2str(attribcol2(1:numcol)) ']']);
      | 	set_param(gcb, 'attribcol3', ['[' num2str(attribcol3(1:numcol)) ']']);
      | 	set_param(gcb, 'attribcol4', ['[' num2str(attribcol4(1:numcol)) ']']);
      | end
      mask Callback attribcol4:
      | target_type=get_param(gcb, 'target_type');
      | attribcol1=[str2num(get_param(gcb, 'attribcol1')) 0 0 0 0 0 0];
      | attribcol2=[str2num(get_param(gcb, 'attribcol2')) 0 0 0 0 0 0];
      | attribcol3=[str2num(get_param(gcb, 'attribcol3')) 0 0 0 0 0 0];
      | attribcol4=[str2num(get_param(gcb, 'attribcol4')) 0 0 0 0 0 0];
      | switch target_type(1:3)
      | 	case 'Cir'
      | 		numcol=1;
      | 	case 'Ell'
      | 		numcol=3;
      |     case 'Rec'
      |         numcol=3;
      |     case 'Lin'
      |         numcol=3;
      |     case 'Tri'
      |         numcol=4;
      | 	otherwise
      | 		numcol=1;
      | end
      | if numcol==1
      | 	set_param(gcb, 'attribcol1', num2str(attribcol1(1)));
      | 	set_param(gcb, 'attribcol2', num2str(attribcol2(1)));
      | 	set_param(gcb, 'attribcol3', num2str(attribcol3(1)));
      | 	set_param(gcb, 'attribcol4', num2str(attribcol4(1)));
      | else
      | 	set_param(gcb, 'attribcol1', ['[' num2str(attribcol1(1:numcol)) ']']);
      | 	set_param(gcb, 'attribcol2', ['[' num2str(attribcol2(1:numcol)) ']']);
      | 	set_param(gcb, 'attribcol3', ['[' num2str(attribcol3(1:numcol)) ']']);
      | 	set_param(gcb, 'attribcol4', ['[' num2str(attribcol4(1:numcol)) ']']);
      | end
      mask Display:
      | disp(columntext)
      | port_label('output',1,outputname)
  Matrix Concatenation : Concatenate  NumInputs=4  Mode=Multidimensional array
  Parameter Table Defn : General/Parameter Table Defn  ShowInLibBrowser=0
  Process_Video_CMD : Video/Process_Video_CMD
  "Scope (xPC) " : xpclib/Misc./Scope (xPC)   scopeno=1  scopetype=Target  autostart=on  viewmode=Numerical  formatstr='%15.6f'  grid=on  ylimits=[0,0]  nosamples=250  noprepostsamples=0  interleave=1  triggermode=FreeRun  triggersignal=1  trigsignalfromport=off  triggerlevel=0.0  triggerslope=Either  triggerscope=1  triggersample=0  filename=data.dat  mode=Lazy  writesize=512  autorestart=off  dynamicfilemode=off  maxwritefilesize=512*1024^2
  Show_Midline_Target : Subsystem  AncestorBlock=Video/Show_Target  mask(Show_Target){target_type=Circle, num_states=1, attribcol1=[6 6 0 3], attribcol2=[6 6 0 3], attribcol3=[7 7 0 3], attribcol4=[8 8 0 3], attribcol5=[0 0 24 0], stateindices_padding=[0 0 0 0 0 0 0;0 0 0 0 0 0 0;0 0 0 0 0 0 0;0 0 0 0 0 0 0;0 0 0 0 0 0 0], source=internal, opacity=100, target_display=Both subject and operator displays}
      mask prompts: target_type "Type of Target"; num_states "Number of Target States"; attribcol1 "State 1 Target Table Column(s)"; attribcol2 "State 2 Target Table Column(s)"; attribcol3 "State 3 Target Table Column(s)"; attribcol4 "State 4 Target Table Column(s)"; attribcol5 "State 5 Target Table Column(s)"; stateindices_padding "State Indices Padding"; source "Source for Opacity"; target_display "Target Display"
      mask help: This block returns a VCODE that, when sent to the Process_Video_CMD block, will cause a single target to be drawn. Target parameters are specified in the Target Table according to the columns defined below and the row input to this block.
      mask init:
      | block_path = gcb;  % store block path, as gcb may change with block operations
      | 
      | % Handle background colours if link status changes.  If the link is resolved, 
      | % make the block back to the library colour.  If the link is not resolved, 
      | % change the colour to something other than the library block colour (but 
      | % only change it if it is the library colour, that way end-users can choose
      | % their own colour.
      | link_status = get_param(block_path, 'LinkStatus');
      | block_parent = get_param(block_path, 'Parent');
      | if strcmp(link_status, 'resolved') || strcmp(block_parent, 'Video')
      | 	set_param(block_path, 'BackgroundColor', '[0.85882, 0.69019, 0.3098]');
      | else
      |  	current_bgcolor = str2num( get_param(block_path, 'BackgroundColor') ) ;
      | 	%if the BackgroundColor is 'green', then after the str2num, current_bgcolor is empty
      | 	if ~isempty(current_bgcolor) 
      | 		if (round(current_bgcolor * 255) == [219 176 79])
      | 	 		set_param(block_path, 'BackgroundColor', 'green');
      | 		end
      | 	end
      | end
      | 
      | num_states=str2num(get_param(gcb, 'num_states'));
      | columntext='';
      | 
      | for i=1:num_states
      | 	varname=['attribcol' num2str(i)];
      | 	if i>1
      | 		columntext=strvcat(columntext, get_param(gcb, varname));
      | 	else
      | 		columntext=[get_param(gcb, varname)];
      | 	end
      | end
      | 
      | space=[''];
      | n=round(length(columntext)/2)-4;
      | for i=1:n
      | 	space=[space ' '];
      | end
      | columntext=strvcat([space '(columns)'], columntext);
      | 
      | output_block=char(find_system(gcb,'LookUnderMasks','all','FollowLinks','on','SearchDepth',1,'BlockType','Outport'));
      | outputname=get_param(output_block,'Name');
      | input_block=find_system(gcb,'LookUnderMasks','all','FollowLinks','on','SearchDepth',1,'BlockType','Inport');
      | inputname1=get_param(char(input_block{1}),'Name');
      | inputname2=get_param(char(input_block{2}),'Name');
      | 
      | if length(input_block) >= 3
      |     inputname3=get_param(char(input_block{3}),'Name');
      | end
      | 
      | source=get_param(gcb,'source');
      | vis=get_param(gcb,'MaskVisibilities');
      | num_states=str2num(get_param(gcb, 'num_states'));
      | 
      | if source=='internal'
      | 	if length(input_block) == 3
      | 		pos=get_param([gcb '/Opacity'],'position');
      | 		delete_line(gcb, 'Opacity/1', 'Embedded MATLAB Function/4');
      | 		delete_block(input_block{3});
      |         add_block('built-in/Constant',[gcb '/Opacity'],'Name','Opacity');
      | 		set_param([gcb '/Opacity'],'position',pos);
      | 		add_line(gcb, 'Opacity/1', 'Embedded MATLAB Function/4');
      | 		set_param([gcb '/Opacity'],'Value','opacity');
      | 	end
      | 	displaytext = ['disp(columntext); port_label(''output'',1,outputname); port_label(''input'',1, inputname1); port_label(''input'',2, inputname2);'];
      | 	vis{10}='on';
      | else
      | 	if length(input_block) == 2
      | 		pos=get_param([gcb '/Opacity'],'position');
      | 		delete_line(gcb, 'Opacity/1', 'Embedded MATLAB Function/4');
      | 		delete_block([gcb, '/Opacity']);
      | 		add_block('built-in/Inport',[gcb '/In2'],'Name','Opacity');
      | 		set_param([gcb '/Opacity'],'position',pos);
      | 		add_line(gcb, 'Opacity/1', 'Embedded MATLAB Function/4');
      |  	end
      | 	inputname3='Opacity';
      | 	displaytext = ['disp(columntext); port_label(''output'',1,outputname); port_label(''input'',1, inputname1); port_label(''input'',2, inputname2); port_label(''input'',3, inputname3);'];
      | 	vis{10}='off';
      | end
      | 
      | targetDisplay = get_param(gcb,'target_display');
      | 
      | if length(targetDisplay) == length('Subject display only')
      |     set_param([gcb '/Target_Display'], 'Value', '2');
      | elseif length(targetDisplay) == length('Operator display only')
      |     set_param([gcb '/Target_Display'], 'Value', '3');
      | else
      |     set_param([gcb '/Target_Display'], 'Value', '1');
      | end
      |     
      | set_param(gcb,'MaskVisibilities',vis);
      | set_param(gcb,'MaskDisplay',displaytext);
      mask Help:
      | Used to draw a single, stationary target.
      | 
      | <H2>Library </H2>
      | Video
      | 
      | <H2>Description </H2>
      | This block returns a VCODE, which when sent to the Process_Video_CMD block will draw a single stationary target.  The VCODE contains all of the target parameters necessary to draw the target.
      | <P>
      | The VCODE is generated from information contained in the Target Table.  Which parts of the Target Table are used depends on the columns selected (see Parameters and Dialog Box below)<P>
      | 
      | <p>For example, assume the "row" input is 2, the "type of target" is set to "Circle" and the "Target Table Columns" is set to [3 0 0 4]. Then using the sample target table below a red circle will be drawn at (20cm, 40cm) and have a radius of 2cm. The zeros in the  "Target Table Columns" indicate those parameters are not used.
      | 
      | <tt>
      | _____________________________________________<br>
      | |&nbsp;&nbsp;&nbsp;&nbsp;&nbsp;&nbsp;&nbsp;&nbsp;&nbsp;&nbsp;| X Pos | Y pos |&nbsp;&nbsp;Fill | Radius |<br>
      | ---------------------------------------------<br>
      | | target 1 |&nbsp;&nbsp;&nbsp;&nbsp;10 |&nbsp;&nbsp;&nbsp;&nbsp;10 | white |&nbsp;&nbsp;&nbsp;&nbsp;&nbsp;&nbsp;5 |<br>
      | | target 2 |&nbsp;&nbsp;&nbsp;&nbsp;20 |&nbsp;&nbsp;&nbsp;&nbsp;40 |&nbsp;&nbsp;&nbsp;red |&nbsp;&nbsp;&nbsp;&nbsp;&nbsp;&nbsp;2 |<br>
      | | target 3 |&nbsp;&nbsp;&nbsp;-40 |&nbsp;&nbsp;&nbsp;&nbsp;10 |&nbsp;&nbsp;blue |&nbsp;&nbsp;&nbsp;&nbsp;&nbsp;&nbsp;3 |<br>
      | ---------------------------------------------<br>
      | </tt>
      | <p> Inputs:<br>
      | <B> Target_Row: </B> this scalar input determines which row in the Target Table is used to define the target parameters.  Typically the Target_Row comes from the Trial_Protocol.  <P>
      | <B> Target_State: </B> this scalar input determines which state the Target is in.  Different states reference different columns in the Target Table (as defined in the Dialog Box).  Typically the Target_State is controlled by the Stateflow_chart to dynamically change the appearance of the target depending on system and/or subject behavior.  Target_State=0 is a valid input, which turns the target off (the intended method for turning a target off is to set Target_State=0). <BR>
      | <P>
      | There is one output from this block:
      | <P>
      | <B> VCODE: </B> this output is a vector containing one VCODE.  This output must go to the Process_Video_CMD block of the video library for the target to actually be shown (if any other visual targets are to be displayed, then this VCODE output must be concatenated with the other VCODES prior to connection to the Process_Video_CMD block - see Help for the Process_Video_CMD block for more information).
      | <P>
      | To show multiple targets simultaneously, multiple copies of the Show_Target block can be used in a Task Program.  The output VCODES from multiple Show_Target blocks must be concatenated prior to connection to the Process_Video_CMD block.
      | <P>
      | 
      | <H2>Parameters and Dialog Box</H2>
      | <B>Type of Target:</B> Choose the type of target specified in the target table.
      | <P>
      | <B>Number of Target States:</B> Choose the number of target states specified in each target row.  Up to five target states are allowed per target row.
      | <P>
      | <B>State [n] Target Table Columns:</B> Enter the column indices that specify the relevant target attributes in the Target Table.  All target types have the same first three target attributes: fill colour, stroke colour and stroke width.
      | <Blockquote>
      | <P>
      | Element 1 (fill colour) - points to the column index in the Target Table containing the fill colour.  If this index is 0, then the fill colour is transparent and the Target Table is not referenced.  For line targets, the fill colour is not used.
      | <P>
      | Element 2 (stroke colour) - points to the column index in the Target Table containing the stroke colour.  If this index is 0, then the stroke colour is transparent and the Target Table is not referenced.  It is possible to use the same column index for both fill colour and stroke colour (i.e.  if single-colour targets are desired).  For line targets, stroke colour defines the colour of the line.
      | <P>
      | Element 3 (stroke width) - points to the column index in the Target Table containing the stroke width (cm).  If no stroke is desired, then setting the stroke column index to 0 will produce a stroke width of 0  and the Target Table is not referenced.  Setting stroke column index to a value less than;0 will produce a standard 1 mm stroke width, again without referencing the Target Table.  For line targets, stroke width defines the width of the line.
      | <P>
      | <B><I>Circle</I></B> <P>
      | Element 4 (radius) - radius of the circle (cm).
      | <P>
      | <B><I>Ellipse</I></B> <P>
      | Elements 4-6 (ellipse properties) - major radius (cm), minor radius (cm), rotation angle (degrees).  If no rotation is desired, then setting rotation column index to 0 will produce a default rotation of 0 and the Target Table will not be referenced.
      | <P>
      | <B><I>Rectangle</I></B><P>
      | Elements 4-6 (rectangle properties) - length (cm), height (cm), rotation angle (degrees).  If no rotation is desired, then setting rotation column index to 0 will produce a default rotation of 0 and the Target Table will not be referenced.
      | <P>
      | <B><I>Line</I></B><P>
      | Elements 4-5 (line properties) - end point x-axis position relative to start point (cm), end point y-axis position relative to start point (cm). The width and colour of the line are defined by the stroke width and the stroke colour, respectively.  The fill colour column is ignored (i.e. any value can be used for column 1)
      | <P>
      | <B><I>Triangle</I></B><P>
      | Elements 4-7 (triangle properties) - length (cm), height (cm), offset of peak of triangle relative to midpoint of the length (cm), rotation angle (degrees). If a height column index of 0 is specified, then an equilateral triangle with sides of the specified length will be created and the Target Table will not be referenced for height or peak offset.  If no rotation is desired, then setting a rotation column index of 0 will produce a default rotation of 0 and the Target Table will not be referenced.
      | </Blockquote>
      | <P>
      | Each target state requires its own set of column index definitions (although multiple states can point to the same column index if desired).<P>
      | <H2>Examples</H2>
      | <B>Example 1.</B>  Suppose a target row will be used to define 2 states for a circle type target.  The first state will be a solid circle of colour1 and the second state will be identical, except that it will have colour2.  The related Target Table columns are: column 4 = colour1; column 5 = colour2 and column 6 = radius.  For this example, "State 1 Target Table Columns" would equal [4 4 0 6], while "State 2 Target Table Columns" would equal [5 5 0 6].  In other words, the fill and stroke colours are both taken from the same column of the Target Table, and there is no outside stroke.
      | <P>
      | 
      | <B>Example 2.</B>  Suppose a target row will be used to define 2 states for an circle type target.  The first state will have fill colour "colour1" and stroke colour "colour2" and radius "rad1".  The second state will have fill colour "colour3" and stroke colour "colour2" and radius "rad2".  Both states will have stroke width "str_width".  The related Target Table columns are: column4 = colour1; column 5 = colour2; column 6 = colour3; column 7 = str_width; column 8 = rad1; column 9 = rad2.  For this example, "State 1 Target Table Columns" would equal [4 5 7 8], while "State 2 Target Table Columns" would equal [6 5 7 9].
      | <P>
      | 
      | <B>Example 3.</B>  Suppose a target row will be used to define 1 state for an ellipse type target.  It will be an outline ellipse with a stroke colour but no fill colour and a standard 1mm stroke width.  The related Target Table columns are: column 4 = colour; column 5 = major radius; column 6 = minor radius and column 7 = orientation.  For this example, "State 1 Target Table Columns" would equal [0 4 -1 5 6 7].
      | <P>
      | 
      | <H2>Related Blocks </H2>
      | Show_Target_With_Label<BR>
      | Process_Video_CMD
      mask TypeOptions target_type: Circle | Ellipse | Rectangle | Line | Triangle
      mask Callback target_type:
      | target_type=get_param(gcb, 'target_type');
      | attribcol1=[str2num(get_param(gcb, 'attribcol1')) 0 0 0 0 0 0];
      | attribcol2=[str2num(get_param(gcb, 'attribcol2')) 0 0 0 0 0 0];
      | attribcol3=[str2num(get_param(gcb, 'attribcol3')) 0 0 0 0 0 0];
      | attribcol4=[str2num(get_param(gcb, 'attribcol4')) 0 0 0 0 0 0];
      | attribcol5=[str2num(get_param(gcb, 'attribcol5')) 0 0 0 0 0 0];
      | switch target_type(1:3)
      | 	case 'Cir'
      | 		numcol=4;
      | 	case 'Ell'
      | 		numcol=6;
      |     case 'Rec'
      |         numcol=6;
      |     case 'Lin'
      |         numcol=5;
      |     case 'Tri'
      |         numcol=7;
      |     otherwise
      | 		numcol=4;
      | end
      | set_param(gcb, 'attribcol1', mat2str(attribcol1(1:numcol)));
      | set_param(gcb, 'attribcol2', mat2str(attribcol2(1:numcol)));
      | set_param(gcb, 'attribcol3', mat2str(attribcol3(1:numcol)));
      | set_param(gcb, 'attribcol4', mat2str(attribcol4(1:numcol)));
      | set_param(gcb, 'attribcol5', mat2str(attribcol5(1:numcol)));
      | 
      | stateindices_padding=zeros(5,7);
      | set_param(gcb, 'stateindices_padding', mat2str(stateindices_padding(:, 1:(11-numcol))));
      mask TypeOptions num_states: 1 | 2 | 3 | 4 | 5
      mask Callback num_states:
      | main_block=gcb;
      | num_states=str2num(get_param(main_block, 'num_states'));
      | vis=get_param(main_block,'MaskVisibilities');
      | 
      | %If the number of states>1, then output an array instead of a vector.
      | %Only show those inputs necessary on the Mask
      | output_block=char(find_system(gcb,'LookUnderMasks','all','SearchDepth',1,'BlockType','Outport'));
      | if num_states==1			%output of HandInTarget block is a vector
      | 	vis{4}='off';
      | 	vis{5}='off';
      | 	vis{6}='off';
      | 	vis{7}='off';
      | elseif num_states==2					%output of HandInTarget block is an array
      | 	vis{4}='on';
      | 	vis{5}='off';
      | 	vis{6}='off';
      | 	vis{7}='off';
      | elseif num_states==3					%output of HandInTarget block is an array
      | 	vis{4}='on';
      | 	vis{5}='on';
      | 	vis{6}='off';
      | 	vis{7}='off';
      | elseif num_states==4					%output of HandInTarget block is an array
      | 	vis{4}='on';
      | 	vis{5}='on';
      | 	vis{6}='on';
      | 	vis{7}='off';
      | else								%output of HandInTarget block is an array
      | 	vis{4}='on';
      | 	vis{5}='on';
      | 	vis{6}='on';
      | 	vis{7}='on';
      | end
      | set_param(main_block,'MaskVisibilities',vis);
      | 
      | target_type=get_param(gcb, 'target_type');
      | attribcol1=[str2num(get_param(gcb, 'attribcol1')) 0 0 0 0 0 0];
      | attribcol2=[str2num(get_param(gcb, 'attribcol2')) 0 0 0 0 0 0];
      | attribcol3=[str2num(get_param(gcb, 'attribcol3')) 0 0 0 0 0 0];
      | attribcol4=[str2num(get_param(gcb, 'attribcol4')) 0 0 0 0 0 0];
      | attribcol5=[str2num(get_param(gcb, 'attribcol5')) 0 0 0 0 0 0];
      | switch target_type(1:3)
      | 	case 'Cir'
      | 		numcol=4;
      | 	case 'Ell'
      | 		numcol=6;
      |     case 'Rec'
      |         numcol=6;
      |     case 'Lin'
      |         numcol=5;
      |     case 'Tri'
      |         numcol=7;
      |     otherwise
      | 		numcol=4;
      | end
      | set_param(gcb, 'attribcol1', mat2str(attribcol1(1:numcol)));
      | set_param(gcb, 'attribcol2', mat2str(attribcol2(1:numcol)));
      | set_param(gcb, 'attribcol3', mat2str(attribcol3(1:numcol)));
      | set_param(gcb, 'attribcol4', mat2str(attribcol4(1:numcol)));
      | set_param(gcb, 'attribcol5', mat2str(attribcol5(1:numcol)));
      | 
      | stateindices_padding=zeros(5,7);
      | set_param(gcb, 'stateindices_padding', mat2str(stateindices_padding(:, 1:(11-numcol))));
      mask Callback attribcol1:
      | target_type=get_param(gcb, 'target_type');
      | attribcol1=[str2num(get_param(gcb, 'attribcol1')) 0 0 0 0 0 0];
      | attribcol2=[str2num(get_param(gcb, 'attribcol2')) 0 0 0 0 0 0];
      | attribcol3=[str2num(get_param(gcb, 'attribcol3')) 0 0 0 0 0 0];
      | attribcol4=[str2num(get_param(gcb, 'attribcol4')) 0 0 0 0 0 0];
      | attribcol5=[str2num(get_param(gcb, 'attribcol5')) 0 0 0 0 0 0];
      | switch target_type(1:3)
      | 	case 'Cir'
      | 		numcol=4;
      | 	case 'Ell'
      | 		numcol=6;
      |     case 'Rec'
      |         numcol=6;
      |     case 'Lin'
      |         numcol=5;
      |     case 'Tri'
      |         numcol=7;
      |     otherwise
      | 		numcol=4;
      | end
      | set_param(gcb, 'attribcol1', mat2str(attribcol1(1:numcol)));
      | set_param(gcb, 'attribcol2', mat2str(attribcol2(1:numcol)));
      | set_param(gcb, 'attribcol3', mat2str(attribcol3(1:numcol)));
      | set_param(gcb, 'attribcol4', mat2str(attribcol4(1:numcol)));
      | set_param(gcb, 'attribcol5', mat2str(attribcol5(1:numcol)));
      | 
      | stateindices_padding=zeros(5,7);
      | set_param(gcb, 'stateindices_padding', mat2str(stateindices_padding(:, 1:(11-numcol))));
      mask Callback attribcol2:
      | target_type=get_param(gcb, 'target_type');
      | attribcol1=[str2num(get_param(gcb, 'attribcol1')) 0 0 0 0 0 0];
      | attribcol2=[str2num(get_param(gcb, 'attribcol2')) 0 0 0 0 0 0];
      | attribcol3=[str2num(get_param(gcb, 'attribcol3')) 0 0 0 0 0 0];
      | attribcol4=[str2num(get_param(gcb, 'attribcol4')) 0 0 0 0 0 0];
      | attribcol5=[str2num(get_param(gcb, 'attribcol5')) 0 0 0 0 0 0];
      | switch target_type(1:3)
      | 	case 'Cir'
      | 		numcol=4;
      | 	case 'Ell'
      | 		numcol=6;
      |     case 'Rec'
      |         numcol=6;
      |     case 'Lin'
      |         numcol=5;
      |     case 'Tri'
      |         numcol=7;
      |     otherwise
      | 		numcol=4;
      | end
      | set_param(gcb, 'attribcol1', mat2str(attribcol1(1:numcol)));
      | set_param(gcb, 'attribcol2', mat2str(attribcol2(1:numcol)));
      | set_param(gcb, 'attribcol3', mat2str(attribcol3(1:numcol)));
      | set_param(gcb, 'attribcol4', mat2str(attribcol4(1:numcol)));
      | set_param(gcb, 'attribcol5', mat2str(attribcol5(1:numcol)));
      | 
      | stateindices_padding=zeros(5,7);
      | set_param(gcb, 'stateindices_padding', mat2str(stateindices_padding(:, 1:(11-numcol))));
      mask Callback attribcol3:
      | target_type=get_param(gcb, 'target_type');
      | attribcol1=[str2num(get_param(gcb, 'attribcol1')) 0 0 0 0 0 0];
      | attribcol2=[str2num(get_param(gcb, 'attribcol2')) 0 0 0 0 0 0];
      | attribcol3=[str2num(get_param(gcb, 'attribcol3')) 0 0 0 0 0 0];
      | attribcol4=[str2num(get_param(gcb, 'attribcol4')) 0 0 0 0 0 0];
      | attribcol5=[str2num(get_param(gcb, 'attribcol5')) 0 0 0 0 0 0];
      | switch target_type(1:3)
      | 	case 'Cir'
      | 		numcol=4;
      | 	case 'Ell'
      | 		numcol=6;
      |     case 'Rec'
      |         numcol=6;
      |     case 'Lin'
      |         numcol=5;
      |     case 'Tri'
      |         numcol=7;
      |     otherwise
      | 		numcol=4;
      | end
      | set_param(gcb, 'attribcol1', mat2str(attribcol1(1:numcol)));
      | set_param(gcb, 'attribcol2', mat2str(attribcol2(1:numcol)));
      | set_param(gcb, 'attribcol3', mat2str(attribcol3(1:numcol)));
      | set_param(gcb, 'attribcol4', mat2str(attribcol4(1:numcol)));
      | set_param(gcb, 'attribcol5', mat2str(attribcol5(1:numcol)));
      | 
      | stateindices_padding=zeros(5,7);
      | set_param(gcb, 'stateindices_padding', mat2str(stateindices_padding(:, 1:(11-numcol))));
      mask Callback attribcol4:
      | target_type=get_param(gcb, 'target_type');
      | attribcol1=[str2num(get_param(gcb, 'attribcol1')) 0 0 0 0 0 0];
      | attribcol2=[str2num(get_param(gcb, 'attribcol2')) 0 0 0 0 0 0];
      | attribcol3=[str2num(get_param(gcb, 'attribcol3')) 0 0 0 0 0 0];
      | attribcol4=[str2num(get_param(gcb, 'attribcol4')) 0 0 0 0 0 0];
      | attribcol5=[str2num(get_param(gcb, 'attribcol5')) 0 0 0 0 0 0];
      | switch target_type(1:3)
      | 	case 'Cir'
      | 		numcol=4;
      | 	case 'Ell'
      | 		numcol=6;
      |     case 'Rec'
      |         numcol=6;
      |     case 'Lin'
      |         numcol=5;
      |     case 'Tri'
      |         numcol=7;
      |     otherwise
      | 		numcol=4;
      | end
      | set_param(gcb, 'attribcol1', mat2str(attribcol1(1:numcol)));
      | set_param(gcb, 'attribcol2', mat2str(attribcol2(1:numcol)));
      | set_param(gcb, 'attribcol3', mat2str(attribcol3(1:numcol)));
      | set_param(gcb, 'attribcol4', mat2str(attribcol4(1:numcol)));
      | set_param(gcb, 'attribcol5', mat2str(attribcol5(1:numcol)));
      | 
      | stateindices_padding=zeros(5,7);
      | set_param(gcb, 'stateindices_padding', mat2str(stateindices_padding(:, 1:(11-numcol))));
      mask Callback attribcol5:
      | target_type=get_param(gcb, 'target_type');
      | attribcol1=[str2num(get_param(gcb, 'attribcol1')) 0 0 0 0 0 0];
      | attribcol2=[str2num(get_param(gcb, 'attribcol2')) 0 0 0 0 0 0];
      | attribcol3=[str2num(get_param(gcb, 'attribcol3')) 0 0 0 0 0 0];
      | attribcol4=[str2num(get_param(gcb, 'attribcol4')) 0 0 0 0 0 0];
      | attribcol5=[str2num(get_param(gcb, 'attribcol5')) 0 0 0 0 0 0];
      | switch target_type(1:3)
      | 	case 'Cir'
      | 		numcol=4;
      | 	case 'Ell'
      | 		numcol=6;
      |     case 'Rec'
      |         numcol=6;
      |     case 'Lin'
      |         numcol=5;
      |     case 'Tri'
      |         numcol=7;
      |     otherwise
      | 		numcol=4;
      | end
      | set_param(gcb, 'attribcol1', mat2str(attribcol1(1:numcol)));
      | set_param(gcb, 'attribcol2', mat2str(attribcol2(1:numcol)));
      | set_param(gcb, 'attribcol3', mat2str(attribcol3(1:numcol)));
      | set_param(gcb, 'attribcol4', mat2str(attribcol4(1:numcol)));
      | set_param(gcb, 'attribcol5', mat2str(attribcol5(1:numcol)));
      | 
      | stateindices_padding=zeros(5,7);
      | set_param(gcb, 'stateindices_padding', mat2str(stateindices_padding(:, 1:(11-numcol))));
      mask TypeOptions source: internal | external
      mask TypeOptions target_display: Both subject and operator displays | Subject display only | Operator display only
      mask Display: disp(columntext); port_label('output',1,outputname); port_label('input',1, inputname1); port_label('input',2, inputname2);
  Show_Mirror_Target : Subsystem  AncestorBlock=Video/Show_Target  mask(Show_Target){target_type=Circle, num_states=1, attribcol1=[6 6 0 3], attribcol2=[6 6 0 3], attribcol3=[7 7 0 3], attribcol4=[8 8 0 3], attribcol5=[0 0 24 0], stateindices_padding=[0 0 0 0 0 0 0;0 0 0 0 0 0 0;0 0 0 0 0 0 0;0 0 0 0 0 0 0;0 0 0 0 0 0 0], source=internal, opacity=100, target_display=Both subject and operator displays}
      mask prompts: target_type "Type of Target"; num_states "Number of Target States"; attribcol1 "State 1 Target Table Column(s)"; attribcol2 "State 2 Target Table Column(s)"; attribcol3 "State 3 Target Table Column(s)"; attribcol4 "State 4 Target Table Column(s)"; attribcol5 "State 5 Target Table Column(s)"; stateindices_padding "State Indices Padding"; source "Source for Opacity"; target_display "Target Display"
      mask help: This block returns a VCODE that, when sent to the Process_Video_CMD block, will cause a single target to be drawn. Target parameters are specified in the Target Table according to the columns defined below and the row input to this block.
      mask init: same as bimanual_Diedrichsen/Show_Midline_Target
      mask Help:
      | Used to draw a single, stationary target.
      | 
      | <H2>Library </H2>
      | Video
      | 
      | <H2>Description </H2>
      | This block returns a VCODE, which when sent to the Process_Video_CMD block will draw a single stationary target.  The VCODE contains all of the target parameters necessary to draw the target.
      | <P>
      | The VCODE is generated from information contained in the Target Table.  Which parts of the Target Table are used depends on the columns selected (see Parameters and Dialog Box below)<P>
      | 
      | <p>For example, assume the "row" input is 2, the "type of target" is set to "Circle" and the "Target Table Columns" is set to [3 0 0 4]. Then using the sample target table below a red circle will be drawn at (20cm, 40cm) and have a radius of 2cm. The zeros in the  "Target Table Columns" indicate those parameters are not used.
      | 
      | <tt>
      | _____________________________________________<br>
      | |&nbsp;&nbsp;&nbsp;&nbsp;&nbsp;&nbsp;&nbsp;&nbsp;&nbsp;&nbsp;| X Pos | Y pos |&nbsp;&nbsp;Fill | Radius |<br>
      | ---------------------------------------------<br>
      | | target 1 |&nbsp;&nbsp;&nbsp;&nbsp;10 |&nbsp;&nbsp;&nbsp;&nbsp;10 | white |&nbsp;&nbsp;&nbsp;&nbsp;&nbsp;&nbsp;5 |<br>
      | | target 2 |&nbsp;&nbsp;&nbsp;&nbsp;20 |&nbsp;&nbsp;&nbsp;&nbsp;40 |&nbsp;&nbsp;&nbsp;red |&nbsp;&nbsp;&nbsp;&nbsp;&nbsp;&nbsp;2 |<br>
      | | target 3 |&nbsp;&nbsp;&nbsp;-40 |&nbsp;&nbsp;&nbsp;&nbsp;10 |&nbsp;&nbsp;blue |&nbsp;&nbsp;&nbsp;&nbsp;&nbsp;&nbsp;3 |<br>
      | ---------------------------------------------<br>
      | </tt>
      | <p> Inputs:<br>
      | <B> Target_Row: </B> this scalar input determines which row in the Target Table is used to define the target parameters.  Typically the Target_Row comes from the Trial_Protocol.  <P>
      | <B> Target_State: </B> this scalar input determines which state the Target is in.  Different states reference different columns in the Target Table (as defined in the Dialog Box).  Typically the Target_State is controlled by the Stateflow_chart to dynamically change the appearance of the target depending on system and/or subject behavior.  Target_State=0 is a valid input, which turns the target off (the intended method for turning a target off is to set Target_State=0). <BR>
      | <P>
      | There is one output from this block:
      | <P>
      | <B> VCODE: </B> this output is a vector containing one VCODE.  This output must go to the Process_Video_CMD block of the video library for the target to actually be shown (if any other visual targets are to be displayed, then this VCODE output must be concatenated with the other VCODES prior to connection to the Process_Video_CMD block - see Help for the Process_Video_CMD block for more information).
      | <P>
      | To show multiple targets simultaneously, multiple copies of the Show_Target block can be used in a Task Program.  The output VCODES from multiple Show_Target blocks must be concatenated prior to connection to the Process_Video_CMD block.
      | <P>
      | 
      | <H2>Parameters and Dialog Box</H2>
      | <B>Type of Target:</B> Choose the type of target specified in the target table.
      | <P>
      | <B>Number of Target States:</B> Choose the number of target states specified in each target row.  Up to five target states are allowed per target row.
      | <P>
      | <B>State [n] Target Table Columns:</B> Enter the column indices that specify the relevant target attributes in the Target Table.  All target types have the same first three target attributes: fill colour, stroke colour and stroke width.
      | <Blockquote>
      | <P>
      | Element 1 (fill colour) - points to the column index in the Target Table containing the fill colour.  If this index is 0, then the fill colour is transparent and the Target Table is not referenced.  For line targets, the fill colour is not used.
      | <P>
      | Element 2 (stroke colour) - points to the column index in the Target Table containing the stroke colour.  If this index is 0, then the stroke colour is transparent and the Target Table is not referenced.  It is possible to use the same column index for both fill colour and stroke colour (i.e.  if single-colour targets are desired).  For line targets, stroke colour defines the colour of the line.
      | <P>
      | Element 3 (stroke width) - points to the column index in the Target Table containing the stroke width (cm).  If no stroke is desired, then setting the stroke column index to 0 will produce a stroke width of 0  and the Target Table is not referenced.  Setting stroke column index to a value less than;0 will produce a standard 1 mm stroke width, again without referencing the Target Table.  For line targets, stroke width defines the width of the line.
      | <P>
      | <B><I>Circle</I></B> <P>
      | Element 4 (radius) - radius of the circle (cm).
      | <P>
      | <B><I>Ellipse</I></B> <P>
      | Elements 4-6 (ellipse properties) - major radius (cm), minor radius (cm), rotation angle (degrees).  If no rotation is desired, then setting rotation column index to 0 will produce a default rotation of 0 and the Target Table will not be referenced.
      | <P>
      | <B><I>Rectangle</I></B><P>
      | Elements 4-6 (rectangle properties) - length (cm), height (cm), rotation angle (degrees).  If no rotation is desired, then setting rotation column index to 0 will produce a default rotation of 0 and the Target Table will not be referenced.
      | <P>
      | <B><I>Line</I></B><P>
      | Elements 4-5 (line properties) - end point x-axis position relative to start point (cm), end point y-axis position relative to start point (cm). The width and colour of the line are defined by the stroke width and the stroke colour, respectively.  The fill colour column is ignored (i.e. any value can be used for column 1)
      | <P>
      | <B><I>Triangle</I></B><P>
      | Elements 4-7 (triangle properties) - length (cm), height (cm), offset of peak of triangle relative to midpoint of the length (cm), rotation angle (degrees). If a height column index of 0 is specified, then an equilateral triangle with sides of the specified length will be created and the Target Table will not be referenced for height or peak offset.  If no rotation is desired, then setting a rotation column index of 0 will produce a default rotation of 0 and the Target Table will not be referenced.
      | </Blockquote>
      | <P>
      | Each target state requires its own set of column index definitions (although multiple states can point to the same column index if desired).<P>
      | <H2>Examples</H2>
      | <B>Example 1.</B>  Suppose a target row will be used to define 2 states for a circle type target.  The first state will be a solid circle of colour1 and the second state will be identical, except that it will have colour2.  The related Target Table columns are: column 4 = colour1; column 5 = colour2 and column 6 = radius.  For this example, "State 1 Target Table Columns" would equal [4 4 0 6], while "State 2 Target Table Columns" would equal [5 5 0 6].  In other words, the fill and stroke colours are both taken from the same column of the Target Table, and there is no outside stroke.
      | <P>
      | 
      | <B>Example 2.</B>  Suppose a target row will be used to define 2 states for an circle type target.  The first state will have fill colour "colour1" and stroke colour "colour2" and radius "rad1".  The second state will have fill colour "colour3" and stroke colour "colour2" and radius "rad2".  Both states will have stroke width "str_width".  The related Target Table columns are: column4 = colour1; column 5 = colour2; column 6 = colour3; column 7 = str_width; column 8 = rad1; column 9 = rad2.  For this example, "State 1 Target Table Columns" would equal [4 5 7 8], while "State 2 Target Table Columns" would equal [6 5 7 9].
      | <P>
      | 
      | <B>Example 3.</B>  Suppose a target row will be used to define 1 state for an ellipse type target.  It will be an outline ellipse with a stroke colour but no fill colour and a standard 1mm stroke width.  The related Target Table columns are: column 4 = colour; column 5 = major radius; column 6 = minor radius and column 7 = orientation.  For this example, "State 1 Target Table Columns" would equal [0 4 -1 5 6 7].
      | <P>
      | 
      | <H2>Related Blocks </H2>
      | Show_Target_With_Label<BR>
      | Process_Video_CMD
      mask TypeOptions target_type: Circle | Ellipse | Rectangle | Line | Triangle
      mask Callback target_type:
      | target_type=get_param(gcb, 'target_type');
      | attribcol1=[str2num(get_param(gcb, 'attribcol1')) 0 0 0 0 0 0];
      | attribcol2=[str2num(get_param(gcb, 'attribcol2')) 0 0 0 0 0 0];
      | attribcol3=[str2num(get_param(gcb, 'attribcol3')) 0 0 0 0 0 0];
      | attribcol4=[str2num(get_param(gcb, 'attribcol4')) 0 0 0 0 0 0];
      | attribcol5=[str2num(get_param(gcb, 'attribcol5')) 0 0 0 0 0 0];
      | switch target_type(1:3)
      | 	case 'Cir'
      | 		numcol=4;
      | 	case 'Ell'
      | 		numcol=6;
      |     case 'Rec'
      |         numcol=6;
      |     case 'Lin'
      |         numcol=5;
      |     case 'Tri'
      |         numcol=7;
      |     otherwise
      | 		numcol=4;
      | end
      | set_param(gcb, 'attribcol1', mat2str(attribcol1(1:numcol)));
      | set_param(gcb, 'attribcol2', mat2str(attribcol2(1:numcol)));
      | set_param(gcb, 'attribcol3', mat2str(attribcol3(1:numcol)));
      | set_param(gcb, 'attribcol4', mat2str(attribcol4(1:numcol)));
      | set_param(gcb, 'attribcol5', mat2str(attribcol5(1:numcol)));
      | 
      | stateindices_padding=zeros(5,7);
      | set_param(gcb, 'stateindices_padding', mat2str(stateindices_padding(:, 1:(11-numcol))));
      mask TypeOptions num_states: 1 | 2 | 3 | 4 | 5
      mask Callback num_states:
      | main_block=gcb;
      | num_states=str2num(get_param(main_block, 'num_states'));
      | vis=get_param(main_block,'MaskVisibilities');
      | 
      | %If the number of states>1, then output an array instead of a vector.
      | %Only show those inputs necessary on the Mask
      | output_block=char(find_system(gcb,'LookUnderMasks','all','SearchDepth',1,'BlockType','Outport'));
      | if num_states==1			%output of HandInTarget block is a vector
      | 	vis{4}='off';
      | 	vis{5}='off';
      | 	vis{6}='off';
      | 	vis{7}='off';
      | elseif num_states==2					%output of HandInTarget block is an array
      | 	vis{4}='on';
      | 	vis{5}='off';
      | 	vis{6}='off';
      | 	vis{7}='off';
      | elseif num_states==3					%output of HandInTarget block is an array
      | 	vis{4}='on';
      | 	vis{5}='on';
      | 	vis{6}='off';
      | 	vis{7}='off';
      | elseif num_states==4					%output of HandInTarget block is an array
      | 	vis{4}='on';
      | 	vis{5}='on';
      | 	vis{6}='on';
      | 	vis{7}='off';
      | else								%output of HandInTarget block is an array
      | 	vis{4}='on';
      | 	vis{5}='on';
      | 	vis{6}='on';
      | 	vis{7}='on';
      | end
      | set_param(main_block,'MaskVisibilities',vis);
      | 
      | target_type=get_param(gcb, 'target_type');
      | attribcol1=[str2num(get_param(gcb, 'attribcol1')) 0 0 0 0 0 0];
      | attribcol2=[str2num(get_param(gcb, 'attribcol2')) 0 0 0 0 0 0];
      | attribcol3=[str2num(get_param(gcb, 'attribcol3')) 0 0 0 0 0 0];
      | attribcol4=[str2num(get_param(gcb, 'attribcol4')) 0 0 0 0 0 0];
      | attribcol5=[str2num(get_param(gcb, 'attribcol5')) 0 0 0 0 0 0];
      | switch target_type(1:3)
      | 	case 'Cir'
      | 		numcol=4;
      | 	case 'Ell'
      | 		numcol=6;
      |     case 'Rec'
      |         numcol=6;
      |     case 'Lin'
      |         numcol=5;
      |     case 'Tri'
      |         numcol=7;
      |     otherwise
      | 		numcol=4;
      | end
      | set_param(gcb, 'attribcol1', mat2str(attribcol1(1:numcol)));
      | set_param(gcb, 'attribcol2', mat2str(attribcol2(1:numcol)));
      | set_param(gcb, 'attribcol3', mat2str(attribcol3(1:numcol)));
      | set_param(gcb, 'attribcol4', mat2str(attribcol4(1:numcol)));
      | set_param(gcb, 'attribcol5', mat2str(attribcol5(1:numcol)));
      | 
      | stateindices_padding=zeros(5,7);
      | set_param(gcb, 'stateindices_padding', mat2str(stateindices_padding(:, 1:(11-numcol))));
      mask Callback attribcol1:
      | target_type=get_param(gcb, 'target_type');
      | attribcol1=[str2num(get_param(gcb, 'attribcol1')) 0 0 0 0 0 0];
      | attribcol2=[str2num(get_param(gcb, 'attribcol2')) 0 0 0 0 0 0];
      | attribcol3=[str2num(get_param(gcb, 'attribcol3')) 0 0 0 0 0 0];
      | attribcol4=[str2num(get_param(gcb, 'attribcol4')) 0 0 0 0 0 0];
      | attribcol5=[str2num(get_param(gcb, 'attribcol5')) 0 0 0 0 0 0];
      | switch target_type(1:3)
      | 	case 'Cir'
      | 		numcol=4;
      | 	case 'Ell'
      | 		numcol=6;
      |     case 'Rec'
      |         numcol=6;
      |     case 'Lin'
      |         numcol=5;
      |     case 'Tri'
      |         numcol=7;
      |     otherwise
      | 		numcol=4;
      | end
      | set_param(gcb, 'attribcol1', mat2str(attribcol1(1:numcol)));
      | set_param(gcb, 'attribcol2', mat2str(attribcol2(1:numcol)));
      | set_param(gcb, 'attribcol3', mat2str(attribcol3(1:numcol)));
      | set_param(gcb, 'attribcol4', mat2str(attribcol4(1:numcol)));
      | set_param(gcb, 'attribcol5', mat2str(attribcol5(1:numcol)));
      | 
      | stateindices_padding=zeros(5,7);
      | set_param(gcb, 'stateindices_padding', mat2str(stateindices_padding(:, 1:(11-numcol))));
      mask Callback attribcol2:
      | target_type=get_param(gcb, 'target_type');
      | attribcol1=[str2num(get_param(gcb, 'attribcol1')) 0 0 0 0 0 0];
      | attribcol2=[str2num(get_param(gcb, 'attribcol2')) 0 0 0 0 0 0];
      | attribcol3=[str2num(get_param(gcb, 'attribcol3')) 0 0 0 0 0 0];
      | attribcol4=[str2num(get_param(gcb, 'attribcol4')) 0 0 0 0 0 0];
      | attribcol5=[str2num(get_param(gcb, 'attribcol5')) 0 0 0 0 0 0];
      | switch target_type(1:3)
      | 	case 'Cir'
      | 		numcol=4;
      | 	case 'Ell'
      | 		numcol=6;
      |     case 'Rec'
      |         numcol=6;
      |     case 'Lin'
      |         numcol=5;
      |     case 'Tri'
      |         numcol=7;
      |     otherwise
      | 		numcol=4;
      | end
      | set_param(gcb, 'attribcol1', mat2str(attribcol1(1:numcol)));
      | set_param(gcb, 'attribcol2', mat2str(attribcol2(1:numcol)));
      | set_param(gcb, 'attribcol3', mat2str(attribcol3(1:numcol)));
      | set_param(gcb, 'attribcol4', mat2str(attribcol4(1:numcol)));
      | set_param(gcb, 'attribcol5', mat2str(attribcol5(1:numcol)));
      | 
      | stateindices_padding=zeros(5,7);
      | set_param(gcb, 'stateindices_padding', mat2str(stateindices_padding(:, 1:(11-numcol))));
      mask Callback attribcol3:
      | target_type=get_param(gcb, 'target_type');
      | attribcol1=[str2num(get_param(gcb, 'attribcol1')) 0 0 0 0 0 0];
      | attribcol2=[str2num(get_param(gcb, 'attribcol2')) 0 0 0 0 0 0];
      | attribcol3=[str2num(get_param(gcb, 'attribcol3')) 0 0 0 0 0 0];
      | attribcol4=[str2num(get_param(gcb, 'attribcol4')) 0 0 0 0 0 0];
      | attribcol5=[str2num(get_param(gcb, 'attribcol5')) 0 0 0 0 0 0];
      | switch target_type(1:3)
      | 	case 'Cir'
      | 		numcol=4;
      | 	case 'Ell'
      | 		numcol=6;
      |     case 'Rec'
      |         numcol=6;
      |     case 'Lin'
      |         numcol=5;
      |     case 'Tri'
      |         numcol=7;
      |     otherwise
      | 		numcol=4;
      | end
      | set_param(gcb, 'attribcol1', mat2str(attribcol1(1:numcol)));
      | set_param(gcb, 'attribcol2', mat2str(attribcol2(1:numcol)));
      | set_param(gcb, 'attribcol3', mat2str(attribcol3(1:numcol)));
      | set_param(gcb, 'attribcol4', mat2str(attribcol4(1:numcol)));
      | set_param(gcb, 'attribcol5', mat2str(attribcol5(1:numcol)));
      | 
      | stateindices_padding=zeros(5,7);
      | set_param(gcb, 'stateindices_padding', mat2str(stateindices_padding(:, 1:(11-numcol))));
      mask Callback attribcol4:
      | target_type=get_param(gcb, 'target_type');
      | attribcol1=[str2num(get_param(gcb, 'attribcol1')) 0 0 0 0 0 0];
      | attribcol2=[str2num(get_param(gcb, 'attribcol2')) 0 0 0 0 0 0];
      | attribcol3=[str2num(get_param(gcb, 'attribcol3')) 0 0 0 0 0 0];
      | attribcol4=[str2num(get_param(gcb, 'attribcol4')) 0 0 0 0 0 0];
      | attribcol5=[str2num(get_param(gcb, 'attribcol5')) 0 0 0 0 0 0];
      | switch target_type(1:3)
      | 	case 'Cir'
      | 		numcol=4;
      | 	case 'Ell'
      | 		numcol=6;
      |     case 'Rec'
      |         numcol=6;
      |     case 'Lin'
      |         numcol=5;
      |     case 'Tri'
      |         numcol=7;
      |     otherwise
      | 		numcol=4;
      | end
      | set_param(gcb, 'attribcol1', mat2str(attribcol1(1:numcol)));
      | set_param(gcb, 'attribcol2', mat2str(attribcol2(1:numcol)));
      | set_param(gcb, 'attribcol3', mat2str(attribcol3(1:numcol)));
      | set_param(gcb, 'attribcol4', mat2str(attribcol4(1:numcol)));
      | set_param(gcb, 'attribcol5', mat2str(attribcol5(1:numcol)));
      | 
      | stateindices_padding=zeros(5,7);
      | set_param(gcb, 'stateindices_padding', mat2str(stateindices_padding(:, 1:(11-numcol))));
      mask Callback attribcol5:
      | target_type=get_param(gcb, 'target_type');
      | attribcol1=[str2num(get_param(gcb, 'attribcol1')) 0 0 0 0 0 0];
      | attribcol2=[str2num(get_param(gcb, 'attribcol2')) 0 0 0 0 0 0];
      | attribcol3=[str2num(get_param(gcb, 'attribcol3')) 0 0 0 0 0 0];
      | attribcol4=[str2num(get_param(gcb, 'attribcol4')) 0 0 0 0 0 0];
      | attribcol5=[str2num(get_param(gcb, 'attribcol5')) 0 0 0 0 0 0];
      | switch target_type(1:3)
      | 	case 'Cir'
      | 		numcol=4;
      | 	case 'Ell'
      | 		numcol=6;
      |     case 'Rec'
      |         numcol=6;
      |     case 'Lin'
      |         numcol=5;
      |     case 'Tri'
      |         numcol=7;
      |     otherwise
      | 		numcol=4;
      | end
      | set_param(gcb, 'attribcol1', mat2str(attribcol1(1:numcol)));
      | set_param(gcb, 'attribcol2', mat2str(attribcol2(1:numcol)));
      | set_param(gcb, 'attribcol3', mat2str(attribcol3(1:numcol)));
      | set_param(gcb, 'attribcol4', mat2str(attribcol4(1:numcol)));
      | set_param(gcb, 'attribcol5', mat2str(attribcol5(1:numcol)));
      | 
      | stateindices_padding=zeros(5,7);
      | set_param(gcb, 'stateindices_padding', mat2str(stateindices_padding(:, 1:(11-numcol))));
      mask TypeOptions source: internal | external
      mask TypeOptions target_display: Both subject and operator displays | Subject display only | Operator display only
      mask Display: disp(columntext); port_label('output',1,outputname); port_label('input',1, inputname1); port_label('input',2, inputname2);
  Show_Target : Video/Show_Target  target_type=Circle  num_states=1  attribcol1=[6 6 0 3]  attribcol2=[6 6 0 3]  attribcol3=[7 7 0 3]  attribcol4=[8 8 0 3]  attribcol5=[0 0 24 0]  stateindices_padding=[0 0 0 0 0 0 0;0 0 0 0 0 0 0;0 0 0 0 0 0 0;0 0 0 0 0 0 0;0 0 0 0 0 0 0]  source=dialog  opacity=100  target_display=Both subject and operator displays  num_col=4
  Sum : Sum  Inputs=|++
  Trial_Control : Stateflow chart  TreatAsAtomicUnit=on
  Velocity_Loads_(2nd hand) : KINARM_EP_loads/Velocity_Loads_EP  use_dom_hand=off  loadcol=[0 2 0 0]  source=dialog  scaling=1  stability=on
  Velocity_Loads_EP : KINARM_EP_loads/Velocity_Loads_EP  use_dom_hand=on  loadcol=[0 1 0 0]  source=dialog  scaling=1  stability=on
  wires:
  Trial_Control/1(logging_enable) -> DataLogging/1
  KINARM_HandInTarget/1 -> Trial_Control/1(HandInTarget)
  Show_Target/1 -> Matrix Concatenation/1
  GUI Control/2 -> Trial_Control/5(Trial_Protocol)
  Trial_Control/8(e_Trial_End) -> GUI Control/1
  GUI Control/1 -> Trial_Control/Trigger
  Trial_Control/5(targetA_state) -> Show_Mirror_Target/2(Target_State), Show_Target/2
  Trial_Control/4(target_row) -> Show_Midline_Target/1(Target_Row), Show_Mirror_Target/1(Target_Row), Show_Target/1
  Matrix Concatenation/1 -> Process_Video_CMD/1
  Trial_Control/7(hand_feedback) -> Custom Hand Feedback/1("feedback_state ")
  Trial_Control/6(targetB_state) -> Show_Midline_Target/2(Target_State)
  KINARM_2ndHandInMirrorTarget/1(HandInTarget_Vector) -> Trial_Control/2(HandIn2ndTarget)
  KINARM_MeanHandInMidlineTarget/1(HandInTarget_Vector) -> Trial_Control/3(HandMeanInTarget)
  GetMeanHandSpeed/1(Out1) -> Trial_Control/4(MeanHandSpeed)
  Show_Mirror_Target/1(VCODE) -> Matrix Concatenation/2
  Show_Midline_Target/1(VCODE) -> Matrix Concatenation/3
  Custom Hand Feedback/1(VCODE) -> Matrix Concatenation/4
  Trial_Control/3(load_row) -> Velocity_Loads_EP/1, Velocity_Loads_(2nd hand)/1
  Trial_Control/2(event_code) -> DataLogging/2
  Velocity_Loads_EP/1 -> Sum/1
  Velocity_Loads_(2nd hand)/1 -> Sum/2
  Forces_to_Torques/1 -> "Scope (xPC) "/1, KINARM_Apply_Loads/1
  Sum/1 -> KINARM_EP_Apply_Loads/1, Forces_to_Torques/1
